simulink model "Chap4_5c"  (R2020b)
settings: Solver=VariableStepAuto  StartTime=0.0  StopTime=10  RelTol=1e-3
StopFcn:
  | Plot4_5c
libraries: simulink_need_slupdate x6
settings Model: Creator=yiyon  LastModifiedBy=yiyon

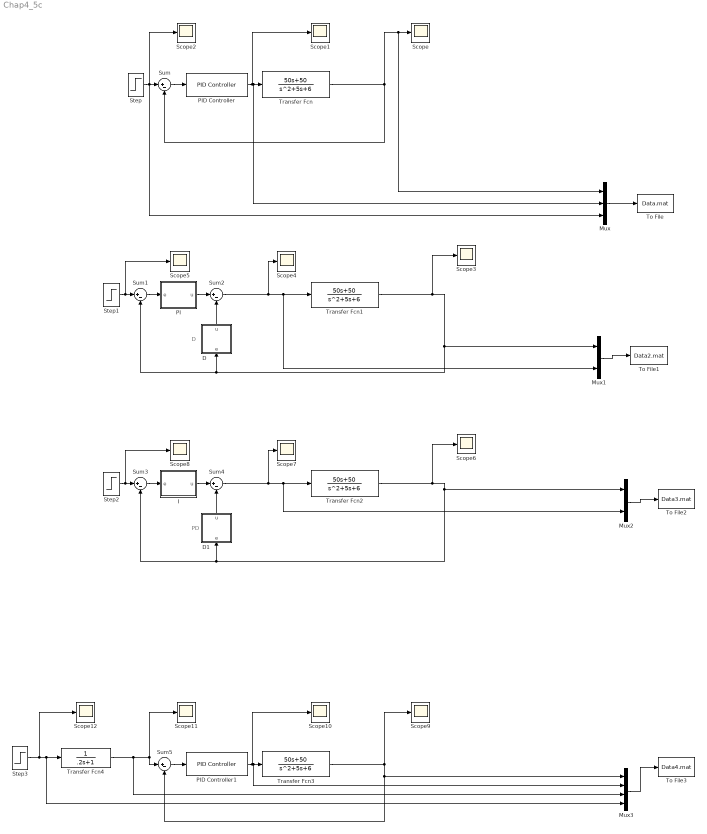
== system Chap4_5c ==
  note: D
  note: PD
  D : Subsystem
  D1 : Subsystem
  I : Subsystem
  Mux : Mux  Inputs=3
  Mux1 : Mux  Inputs=2
  Mux2 : Mux  Inputs=2
  Mux3 : Mux
  PI : Subsystem
  PID Controller : simulink_need_slupdate/PID Controller  P=1.3132  I=0.1637  D=0.0046
  PID Controller1 : simulink_need_slupdate/PID Controller  P=1.3132  I=0.1637  D=0.0046
  Scope{,1..12} (13 alike) : Scope
  Step{,1..3} (4 alike) : Step  Time=2  SampleTime=0
  Sum{,1..5} (6 alike) : Sum  Inputs=|+-  InputSameDT=on  SaturateOnIntegerOverflow=on  OutDataTypeStr=Inherit: Same as first input
  To File : ToFile  Filename=Data.mat  SaveFormat=Timeseries
  To File1 : ToFile  Filename=Data2.mat  SaveFormat=Timeseries
  To File2 : ToFile  Filename=Data3.mat  SaveFormat=Timeseries
  To File3 : ToFile  Filename=Data4.mat  SaveFormat=Timeseries
  Transfer Fcn{,1..3} (4 alike) : TransferFcn  Numerator=[50 50]  Denominator=[1 5 6]
  Transfer Fcn4 : TransferFcn  Denominator=[.2 1]
  wires:
  Step/1 -> Scope2/1, Mux/3, Sum/1
  Transfer Fcn/1 -> Sum/2, Mux/1, Scope/1
  Sum/1 -> PID Controller/1
  PID Controller/1 -> Scope1/1, Mux/2, Transfer Fcn/1
  Mux/1 -> To File/1
  Transfer Fcn1/1 -> Scope3/1, Mux1/1, Sum1/2, D/1(e)
  Step1/1 -> Scope5/1, Sum1/1
  Sum2/1 -> Scope4/1, Mux1/2, Transfer Fcn1/1
  Sum1/1 -> PI/1(e)
  PI/1(u) -> Sum2/1
  D/1(u) -> Sum2/2
  Transfer Fcn2/1 -> Scope6/1, Mux2/1, Sum3/2, D1/1(e)
  Step2/1 -> Scope8/1, Sum3/1
  D1/1(u) -> Sum4/2
  Sum3/1 -> I/1(e)
  I/1(u) -> Sum4/1
  Sum4/1 -> Scope7/1, Mux2/2, Transfer Fcn2/1
  Sum5/1 -> PID Controller1/1
  PID Controller1/1 -> Scope10/1, Mux3/2, Transfer Fcn3/1
  Transfer Fcn3/1 -> Mux3/1, Sum5/2, Scope9/1
  Step3/1 -> Scope12/1, Mux3/4, Transfer Fcn4/1
  Transfer Fcn4/1 -> Mux3/3, Sum5/1, Scope11/1
  Mux1/1 -> To File1/1
  Mux2/1 -> To File2/1
  Mux3/1 -> To File3/1

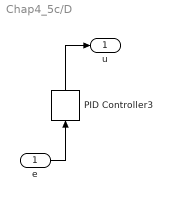
== system Chap4_5c/D ==
  e : Inport
  PID Controller3 : simulink_need_slupdate/PID Controller  P=0  I=0  D=0.0046
  u : Outport
  wires:
  e/1 -> PID Controller3/1
  PID Controller3/1 -> u/1

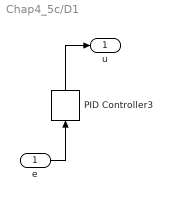
== system Chap4_5c/D1 ==
  e : Inport
  PID Controller3 : simulink_need_slupdate/PID Controller  P=1.3132  I=0  D=0.0046
  u : Outport
  wires:
  e/1 -> PID Controller3/1
  PID Controller3/1 -> u/1

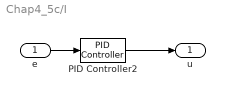
== system Chap4_5c/I ==
  e : Inport
  PID Controller2 : simulink_need_slupdate/PID Controller  P=0  I=0.1637  D=0  mask(PID Controller){}
  u : Outport
  wires:
  e/1 -> PID Controller2/1
  PID Controller2/1 -> u/1

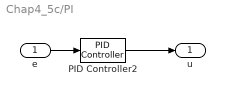
== system Chap4_5c/PI ==
  e : Inport
  PID Controller2 : simulink_need_slupdate/PID Controller  P=1.3132  I=0.1637  D=0  mask(PID Controller){}
  u : Outport
  wires:
  e/1 -> PID Controller2/1
  PID Controller2/1 -> u/1
